simulink model "just_for_pics"  (R2026b)
settings: Solver=FixedStepAuto  StopTime=60  FixedStep=0.01
InitFcn:
  | Calc;
values from neighbouring files (symbols this model uses):
  J = J_r + (J_p/N^2)    (= 0.0035)    [Ches_workspace.m]    (also in linsys1.mat = 0.0396; params.m = 0.0396)
  K_a = 0.2    [Ches_workspace.m]    (also in linsys1.mat; params.m)
  K_b = 0.009549    [Ches_workspace.m]    (also in linsys1.mat; params.m)
  K_f = 0.047746    [Ches_workspace.m]    (also in linsys1.mat; params.m)
  K_p = 4    [Ches_workspace.m]    (also in linsys1.mat; params.m)
  K_s = h*(2/1.8)    (= 1.66666666667)    [Ches_workspace.m]    (also in linsys1.mat = 0.277777777778; params.m = 0.277777777778)
  N = 20    [Ches_workspace.m]    (also in linsys1.mat; params.m)
  R_m = 10    [Ches_workspace.m]    (also in linsys1.mat; params.m)
settings Model: Creator=milan  LastModifiedBy=moore

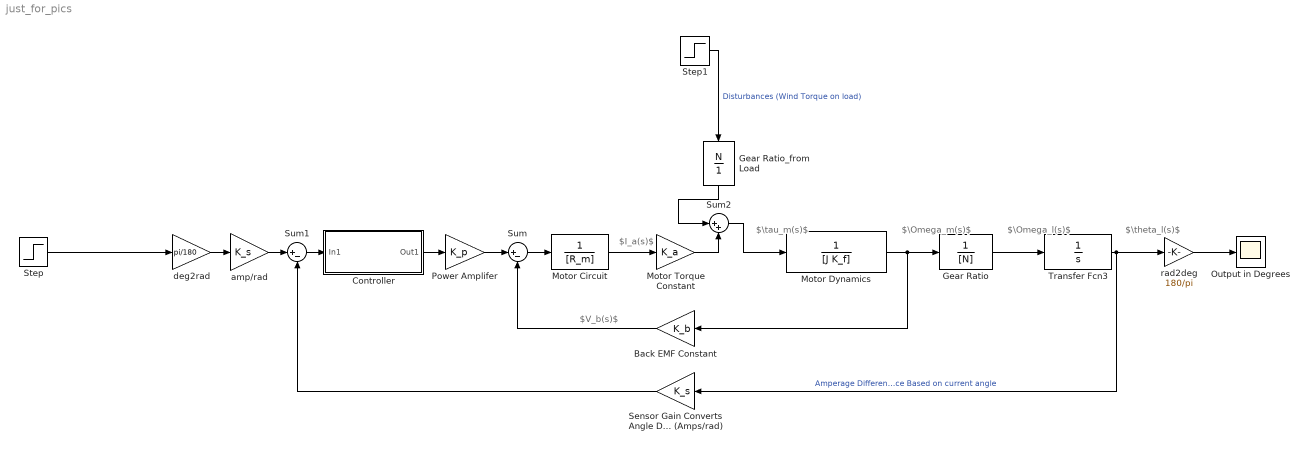
== system just_for_pics ==
  note: $V_b(s)$
  note: $I_a(s)$
  note: $\tau_m(s)$
  note: $\Omega_m(s)$
  note: $\Omega_l(s)$
  note: $\theta_l(s)$
  Back EMF Constant : Gain  Gain=K_b
  Controller : Subsystem
  Gear Ratio : TransferFcn  Denominator=[N]
  Gear Ratio_from Load : TransferFcn  Numerator=N  Denominator=1
  Motor Circuit : TransferFcn  Denominator=[R_m]
  Motor Dynamics : TransferFcn  Denominator=[J K_f]
  Motor Torque Constant : Gain  Gain=K_a
  Output in Degrees : Scope
      settings: ActiveDisplayYMinimum=-7.4761362024830849  ActiveDisplayYMaximum=67.285225822347783
  Power Amplifer : Gain  Gain=K_p
  Sensor Gain Converts Angle Difference into amp difference (Amps/rad) : Gain  Gain=K_s
  Step : Step  Time=0.01  SampleTime=0.01
  Step1 : Step  Time=0.01  SampleTime=0.01
  Sum : Sum  Inputs=|+-
  Sum1 : Sum  Inputs=|+-
  Sum2 : Sum  Inputs=|++
  Transfer Fcn3 : TransferFcn  Denominator=[1 0]
  amp/rad : Gain  Gain=K_s
  deg2rad : Gain  Gain=pi/180
  rad2deg : Gain  Gain=180/pi
  wires:
  Motor Circuit/1 -> Motor Torque Constant/1
  Motor Torque Constant/1 -> Sum2/2
  Motor Dynamics/1 -> Gear Ratio/1, Back EMF Constant/1
  Gear Ratio/1 -> Transfer Fcn3/1
  Transfer Fcn3/1 -> Sensor Gain Converts Angle Difference into amp difference (Amps/rad)/1, rad2deg/1  "Amperage Difference Based on current angle"
  Back EMF Constant/1 -> Sum/2
  Sum/1 -> Motor Circuit/1
  Sensor Gain Converts Angle Difference into amp difference (Amps/rad)/1 -> Sum1/2
  rad2deg/1 -> Output in Degrees/1
  Power Amplifer/1 -> Sum/1
  amp/rad/1 -> Sum1/1
  deg2rad/1 -> amp/rad/1
  Step/1 -> deg2rad/1
  Controller/1(Out1) -> Power Amplifer/1
  Sum1/1 -> Controller/1(In1)
  Sum2/1 -> Motor Dynamics/1
  Gear Ratio_from Load/1 -> Sum2/1
  Step1/1 -> Gear Ratio_from Load/1  "Disturbances (Wind Torque on load)"

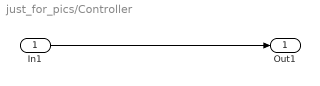
== system just_for_pics/Controller ==
  In1 : Inport
  Out1 : Outport
  wires:
  In1/1 -> Out1/1
